simulink model "TestSupervisorFSM_TX"  (R2025a)
settings: Solver=FixedStepDiscrete  StartTime=0.0  StopTime=inf  RelTol=1e-3  EnableMultiTasking=on
model workspace (MAT data in the model file):
  Command = 1
  State = 0
undefined symbols (not defined in the file): ControlModes
libraries: eeStairGenerator x6
settings Model: DataDictionary=embeddedBoard_common.sldd  Creator=vvasco  LastModifiedBy=mfussi
settings SolverCC: ConcurrentTasks=on  AlgebraicLoopSolver=TrustRegion  AutoInsertRateTranBlk=on
settings DataIOCC: LimitDataPoints=on
settings OptimizationCC: ReuseModelBlockBuffer=off  LifeSpan=inf
settings DebuggingCC: ParameterPrecisionLossMsg=none  UnconnectedInputMsg=warning  UnconnectedOutputMsg=warning  UnconnectedLineMsg=warning  AllowSymbolicDim=off  SFUnexpectedBacktrackingDiag=warning  SFNoUnconditionalDefaultTransitionDiag=warning  SFExecutionAtInitializationDiag=none  ArithmeticOperatorsInVariantConditions=warning
settings ModelReferenceCC: EnableRefExpFcnMdlSchedulingChecks=on
settings SFSimCC: SimUseLocalCustomCode=off  CustomCodeUndefinedFunction=UseInterfaceOnly
settings RTWCC: RTWUseLocalCustomCode=off  GPUComputeCapability=3.5  DLArmComputeVersion=19.05
settings CodeAppCC: StateflowObjectComments=on
settings GRTTargetCC: TargetLangStandard=C89/C90 (ANSI)
settings ConfigComp: CovMetricSettings=dw  CovSaveCumulativeToWorkspaceVar=on  CovSaveSingleToWorkspaceVar=on  CovExternalEMLEnable=off

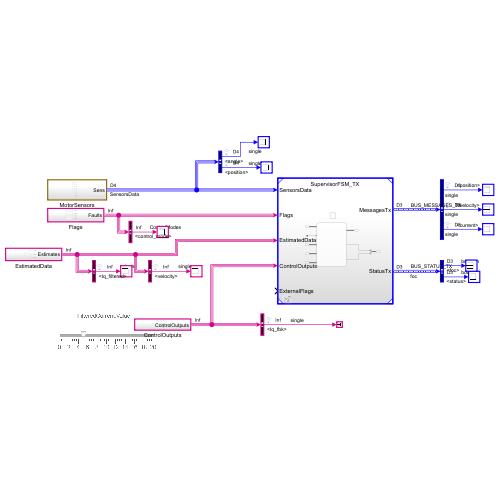
[thumbnail: Simulink's stored preview of the top-level diagram]
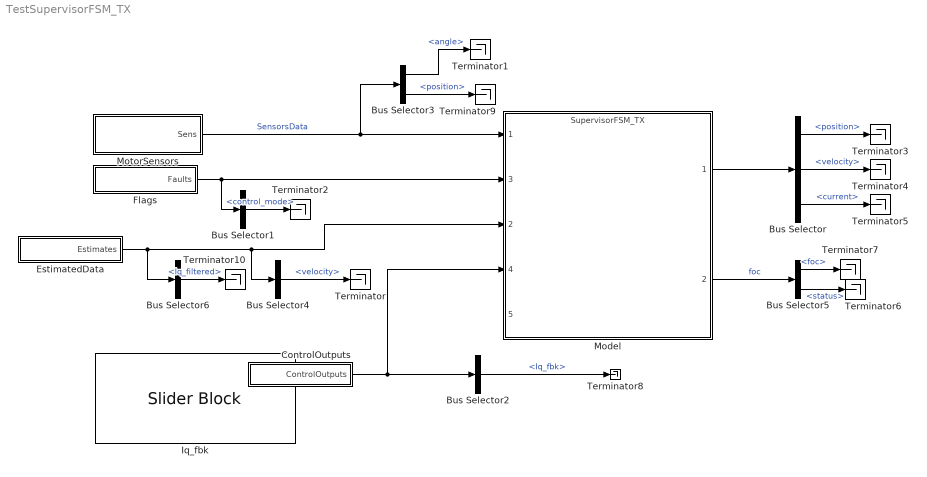
== system TestSupervisorFSM_TX ==
  Bus Selector : BusSelector  OutputSignals=foc.position,foc.velocity,foc.current
  Bus Selector1 : BusSelector  OutputSignals=control_mode
  Bus Selector2 : BusSelector  OutputSignals=Iq_fbk
  Bus Selector3 : BusSelector  OutputSignals=motorsensors.angle,position
  Bus Selector4 : BusSelector  OutputSignals=velocity
  Bus Selector5 : BusSelector  OutputSignals=foc,status
  Bus Selector6 : BusSelector  OutputSignals=Iq_filtered
  ControlOutputs : Subsystem
  EstimatedData : Subsystem
  Flags : Subsystem
  Iq_fbk : SliderBlock  ScaleMax=20
  Model : ModelReference  ModelNameDialog=SupervisorFSM_TX.slx  SimulationMode=Normal  ModelReferenceVersion=10.14
      settings: PortSchema="{\"entries\":[{\"content\":{\"sides\":[{\"content\":{\"connectorIds\":[\"In1\",\"In3\",\"In2\",\"In4\",\"In5\"]},\"type\":\"ConnectorPlacement.EquallySpacedRectSide\",\"uuid\":\"69e4ef43-4003-4440-a894-3828c1af5902\"},{\"content\":{\"connectorIds\":[\"Out1\",\"Out2\"],\"side\":\"RIGHT\"},\"type\":\"ConnectorPlacement.EquallySpacedRectSide\",\"uuid\":\"4c041ecf-670d-4f38-bad4-7d246327a855\"},{\"content\":{\"side\":\"TOP\"},\"type\":\"ConnectorPlacement.EquallySpacedRectSide\",\"uuid\":\"dbbb66c6-d08b-4ab5-92ab-8954eaf6e6e2\"}]},\"type\":\"ConnectorPlacement.EquallySpacedConnector\",\"uuid\":\"4940a0b0-17cd-4df8-8277-6fa028eccbd4\"}],\"packageUris\":[\"http://schema.mathworks.com/mf0/Connector/R2020b\"],\"version\":\"1.0\"}"
  MotorSensors : Subsystem
  Terminator{,1..10} (11 alike) : Terminator
  wires:
  Bus Selector/1 -> Terminator3/1  "<position>"
  Bus Selector3/1 -> Terminator1/1  "<angle>"
  Bus Selector/2 -> Terminator4/1  "<velocity>"
  Bus Selector/3 -> Terminator5/1  "<current>"
  Bus Selector1/1 -> Terminator2/1  "<control_mode>"
  Model/2 -> Bus Selector5/1  "foc"
  Model/1 -> Bus Selector/1
  ControlOutputs/1(ControlOutputs) -> Model/4, Bus Selector2/1
  EstimatedData/1(Estimates) -> Bus Selector6/1, Model/2, Bus Selector4/1
  MotorSensors/1(Sens) -> Model/1, Bus Selector3/1  "SensorsData"
  Bus Selector2/1 -> Terminator8/1  "<Iq_fbk>"
  Bus Selector4/1 -> Terminator/1  "<velocity>"
  Flags/1(Faults) -> Model/3, Bus Selector1/1
  Bus Selector5/1 -> Terminator7/1  "<foc>"
  Bus Selector5/2 -> Terminator6/1  "<status>"
  Bus Selector3/2 -> Terminator9/1  "<position>"
  Bus Selector6/1 -> Terminator10/1  "<Iq_filtered>"

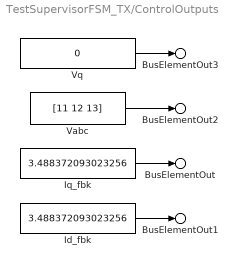
== system TestSupervisorFSM_TX/ControlOutputs ==
  Id_fbk : Constant  Value=3.488372093023256  OutDataTypeStr=single
  Iq_fbk : Constant  Value=3.488372093023256  OutDataTypeStr=single
  Vabc : Constant  Value=[11 12 13]  OutDataTypeStr=single
  Vq : Constant  Value=0  OutDataTypeStr=single
  BusElementOut3 : Outport  Description=control effort (quadrature)  PortName=ControlOutputs  Element=Vq
  BusElementOut2 : Outport  Description=control effort (3-phases)  PortName=ControlOutputs  Element=Vabc
  BusElementOut : Outport  Description=quadrature current  PortName=ControlOutputs  Element=Iq_fbk
  BusElementOut1 : Outport  Description=direct current  PortName=ControlOutputs  Element=Id_fbk
  wires:
  Iq_fbk/1 -> BusElementOut/1
  Id_fbk/1 -> BusElementOut1/1
  Vabc/1 -> BusElementOut2/1
  Vq/1 -> BusElementOut3/1

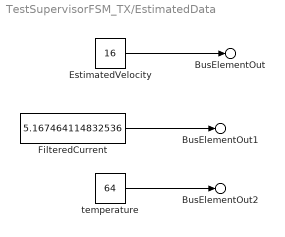
== system TestSupervisorFSM_TX/EstimatedData ==
  EstimatedVelocity : Constant  Value=16  OutDataTypeStr=single
  FilteredCurrent : Constant  Value=5.167464114832536  OutDataTypeStr=single
  temperature : Constant  Value=64  OutDataTypeStr=single
  BusElementOut : Outport  Description=velocity  PortName=Estimates  Element=velocity
  BusElementOut1 : Outport  Description=filtered motor current  PortName=Estimates  Element=Iq_filtered
  BusElementOut2 : Outport  Description=motor temperature  PortName=Estimates  Element=motor_temperature
  wires:
  EstimatedVelocity/1 -> BusElementOut/1
  FilteredCurrent/1 -> BusElementOut1/1
  temperature/1 -> BusElementOut2/1

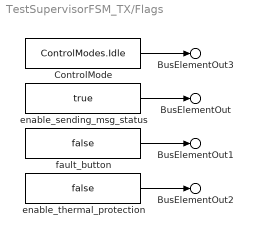
== system TestSupervisorFSM_TX/Flags ==
  ControlMode : Constant  Value=ControlModes.Idle  OutDataTypeStr=Enum: ControlModes
  enable_sending_msg_status : Constant  Value=true  OutDataTypeStr=boolean
  enable_thermal_protection : Constant  Value=false  OutDataTypeStr=boolean
  fault_button : Constant  Value=false  OutDataTypeStr=boolean
  BusElementOut : Outport  PortName=Faults  Element=enable_sending_msg_status
  BusElementOut1 : Outport  PortName=Faults  Element=hw_faults.overcurrent
  BusElementOut2 : Outport  PortName=Faults  Element=enable_thermal_protection
  BusElementOut3 : Outport  Description=control mode  PortName=Faults  Element=control_mode
  wires:
  ControlMode/1 -> BusElementOut3/1
  enable_sending_msg_status/1 -> BusElementOut/1
  fault_button/1 -> BusElementOut1/1
  enable_thermal_protection/1 -> BusElementOut2/1

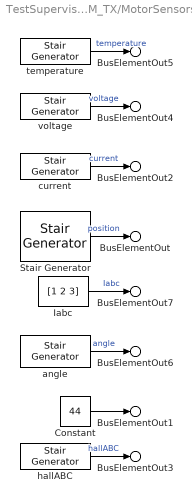
== system TestSupervisorFSM_TX/MotorSensors ==
  Constant : Constant  Value=44  OutDataTypeStr=single  SampleTime=0.1
  Iabc : Constant  Value=[1 2 3]  OutDataTypeStr=single  SampleTime=0.1
  Stair Generator : eeStairGenerator/Stair Generator  LabelModeActiveChoice=Discrete  TimeInput=[0.1 0.2 0.3 0.4 0.5 0.6 0.7 0.8 0.9 1 1.1 1.2 1.3 ]  AmplitudeInput=[20 23 26 29 32 35 38 41 39 36 30 25 20]  SampleTime=0.1  RepeatPattern=on  OutDataTypeStr=single
  angle : eeStairGenerator/Stair Generator  LabelModeActiveChoice=Discrete  TimeInput=[0 1 2 3 4 5 6 7 8 9]  AmplitudeInput=[0 1 6 6 6 1 1 1 2 2]  SampleTime=0.1  RepeatPattern=on  OutDataTypeStr=single
      link override Discrete/Constant: SampleTime=4.5e-05
      link override Discrete/Constant1: SampleTime=-1
      link override Discrete/Constant2: SampleTime=inf
      link override Discrete/Digital Clock: SampleTime=4.5e-05
      link override Discrete/Output: SampleTime=4.5e-05
  current : eeStairGenerator/Stair Generator  LabelModeActiveChoice=Discrete  TimeInput=[0 0.1 0.2 0.3 0.4 0.5 0.6 0.7 0.8 0.9]  AmplitudeInput=[16 10 15 12 10 16 12 16 18 17]  SampleTime=0.1  RepeatPattern=on  OutDataTypeStr=single
  hallABC : eeStairGenerator/Stair Generator  LabelModeActiveChoice=Discrete  TimeInput=[0 0.1 0.2 0.3 0.4 0.5 0.6 0.7 0.8 0.9]  AmplitudeInput=[6 3 5 2 0 6 6 6 6 6]  SampleTime=0.1  RepeatPattern=off  OutDataTypeStr=uint8
  temperature : eeStairGenerator/Stair Generator  LabelModeActiveChoice=Discrete  TimeInput=[0 1 2 3 4 5 6 7 8 9]  AmplitudeInput=[2 2 2 9 9 9 9 9 9 2]  SampleTime=0.1  RepeatPattern=off  OutDataTypeStr=single
  voltage : eeStairGenerator/Stair Generator  LabelModeActiveChoice=Discrete  TimeInput=[0 1 2 3 4 5 6 7 8 9]./10  AmplitudeInput=[2 3 3 3 3 3 2 2 2 2]  SampleTime=0.1  RepeatPattern=on  OutDataTypeStr=single
  BusElementOut : Outport  Description=position encoders  PortName=Sens  Element=position
  BusElementOut1 : Outport  Description=power supply voltage  PortName=Sens  Element=driversensors.Vcc
  BusElementOut7 : Outport  PortName=Sens  Element=motorsensors.Iabc
  BusElementOut6 : Outport  Description=electrical angle = angle * pole_pairs  PortName=Sens  Element=motorsensors.angle
  BusElementOut5 : Outport  PortName=Sens  Element=motorsensors.temperature
  BusElementOut4 : Outport  PortName=Sens  Element=motorsensors.voltage
  BusElementOut2 : Outport  PortName=Sens  Element=motorsensors.current
  BusElementOut3 : Outport  PortName=Sens  Element=motorsensors.hallABC
  wires:
  voltage/1 -> BusElementOut4/1  "voltage"
  temperature/1 -> BusElementOut5/1  "temperature"
  hallABC/1 -> BusElementOut3/1  "hallABC"
  angle/1 -> BusElementOut6/1  "angle"
  current/1 -> BusElementOut2/1  "current"
  Stair Generator/1 -> BusElementOut/1  "position"
  Constant/1 -> BusElementOut1/1
  Iabc/1 -> BusElementOut7/1  "Iabc"
